simulink model "heatdrive_ecc_coupled_se21"  (R2025b)
settings: Solver=ode23t  StartTime=0.0  StopTime=10  FixedStep=0.1  MaxStep=0.4  RelTol=1e-2  AbsTol=1e-3
values from neighbouring files (symbols this model uses):
  cold_load_heat_W = 0.0    (= 0)    [Build_Simulink_Exchange_Params.m]
  cold_load_T_init = get_stage_field(stage_config, 'cold_load_T_in', get_stage_field(stage_config,          'chip_T_in', get_option_field(exchange_options, 'cold_load_T_init', get_option_field(exchange_options, 'chip_T_init', 293.0))))    [Build_Simulink_Exchange_Params.m]    (also in Create_Simulink_Exchange_Runtime.m = get_option_field(options, 'cold_load_T_init',          get_o)
  cold_sink_T_init = get_stage_field(stage_config, 'cold_sink_T_in', get_option_field(exchange_options, 'cold_sink_T_init', 293.0))    [Build_Simulink_Exchange_Params.m]    (also in Create_Simulink_Exchange_Runtime.m = get_option_field(options, 'cold_sink_T_init', ambient_T_init)
  hot_sink_T_init = get_stage_field(stage_config, 'hot_sink_T_in', get_option_field(exchange_options, 'hot_sink_T_init', 293.0))    [Build_Simulink_Exchange_Params.m]    (also in Create_Simulink_Exchange_Runtime.m = get_option_field(options, 'hot_sink_T_init', ambient_T_init))
  mdot_cooldown_source_kgps = mdot_target_kgps    [Build_Simulink_Exchange_Params.m]
  mdot_hold_source_kgps = mdot_target_kgps    [Build_Simulink_Exchange_Params.m]
  pressure_pi_bias_MPa = pressure_pi_dp_guess_MPa    [Build_Simulink_Exchange_Params.m]
  pressure_pi_error_filter_tau_s = max(get_option_field(exchange_options, 'pressure_pi_error_filter_tau_s', 0.002), 1.0e-5)    [Build_Simulink_Exchange_Params.m]
  pressure_pi_error_normalization_gain_kgps_inv = 1.0    (= 1)    [Build_Simulink_Exchange_Params.m]
  pressure_pi_max_MPa = pressure_pi_dp_guess_MPa + pressure_pi_margin_MPa    [Build_Simulink_Exchange_Params.m]
  shex_sink_T_init = get_option_field(exchange_options, 'shex_sink_T_init', hot_sink_T_init)    [Build_Simulink_Exchange_Params.m]
undefined symbols (not defined in the file or in its folder): constitutive_sample_time_s, constitutive_state21_initial, se_constitutive_T21_initial, se_pressure_integrator_max_MPa, se_pressure_pi_ki_MPa_per_kgps_s, se_pressure_pi_kp_MPa_per_kgps, se_pressure_pi_min_MPa, se_solver_T_init_21_internal, se_stage2_pressure_integrator_min_MPa, se_stage4_pressure_integrator_min_MPa, sma_constitutive_T21_initial, sma_mdot_stage1_source_kgps, sma_mdot_stage3_source_kgps, sma_pressure_integrator_max_MPa, sma_pressure_integrator_min_MPa, sma_pressure_pi_ki_MPa_per_kgps_s, sma_pressure_pi_kp_MPa_per_kgps, sma_pressure_pi_min_MPa, sma_solver_T_init_21_internal
libraries: fl_lib x484, nesl_utility x232, SimscapeFluids_lib x20
(part 5 of 8)

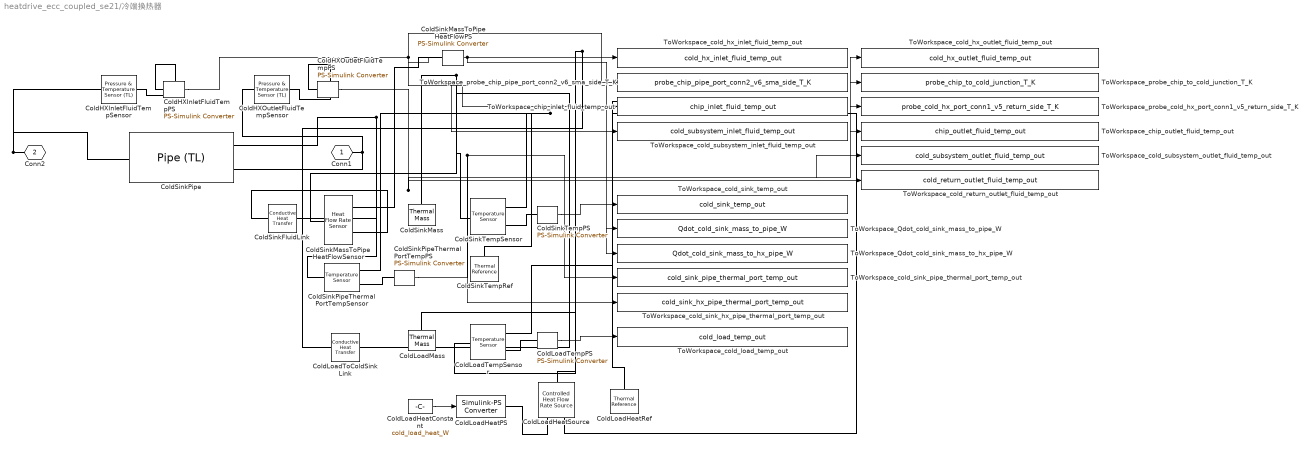
== system heatdrive_ecc_coupled_se21/冷端换热器 ==
  ColdHXInletFluidTempPS : nesl_utility/PS-Simulink Converter  PhysicalDomain=network_engine_domain  SubClassName=ps_output  LeftPortType=input  RightPortType=output  PseudoPeriodic=off  Frequencies=[]  VectorFormat=1-D array  Unit=K  AffineConversion=off
  ColdHXInletFluidTempSensor : fl_lib/Thermal Liquid/Sensors/Pressure & Temperature Sensor (TL)  reference=foundation.enum.MeasurementReference.absolute  pressure=false  pressure_spec=foundation.enum.PressureMeasementSpec.Absolute  temperature=true
      settings: InternalSimscapePortConfiguration="{\"Bottom\":[{\"id\":\"T\",\"label\":\"T\",\"type\":\"output\"}],\"Left\":[{\"id\":\"A\",\"label\":\"A\",\"type\":\"foundation.thermal_liquid.thermal_liquid\"}],\"Right\":[],\"Top\":[]}"
  ColdHXOutletFluidTempPS : nesl_utility/PS-Simulink Converter  PhysicalDomain=network_engine_domain  SubClassName=ps_output  LeftPortType=input  RightPortType=output  PseudoPeriodic=off  Frequencies=[]  VectorFormat=1-D array  Unit=K  AffineConversion=off
  ColdHXOutletFluidTempSensor : fl_lib/Thermal Liquid/Sensors/Pressure & Temperature Sensor (TL)  reference=foundation.enum.MeasurementReference.absolute  pressure=false  pressure_spec=foundation.enum.PressureMeasementSpec.Absolute  temperature=true
      settings: InternalSimscapePortConfiguration="{\"Bottom\":[{\"id\":\"T\",\"label\":\"T\",\"type\":\"output\"}],\"Left\":[{\"id\":\"A\",\"label\":\"A\",\"type\":\"foundation.thermal_liquid.thermal_liquid\"}],\"Right\":[],\"Top\":[]}"
  ColdLoadHeatConstant : Constant  Value=cold_load_heat_W
  ColdLoadHeatPS : nesl_utility/Simulink-PS Converter  PhysicalDomain=network_engine_domain  SubClassName=ps_input  LeftPortType=input  RightPortType=output  PseudoPeriodic=off  Frequencies=[]  NoiseDistribution=none  NoiseParameters=[]  Unit=W  AffineConversion=off  FilteringAndDerivatives=provide  SimscapeFilterOrder=1  InputFilterTimeConstant=0.001  UdotUserProvided=0
  ColdLoadHeatRef : fl_lib/Thermal/Thermal Elements/Thermal Reference
  ColdLoadHeatSource : fl_lib/Thermal/Thermal Sources/Controlled Heat Flow Rate Source
  ColdLoadMass : fl_lib/Thermal/Thermal Elements/Thermal Mass  mass_type=foundation.enum.constant_variable.constant  mass=cold_load_mass_kg kg  sp_heat=thermal_mass_cp_ref J/(K*kg)  mass_min=1e-6 kg  num_ports=foundation.enum.numPorts2.one  m_specify=off  m_priority=High  m=1 kg  m_nominal_specify=off  m_nominal_value=1  m_nominal_unit=kg  T_specify=on  T_priority=High  T=cold_load_T_init K  T_nominal_specify=off  T_nominal_value=1  T_nominal_unit=K  Q_specify=off  Q_priority=None  Q=0 W  Q_nominal_specify=off  Q_nominal_value=1  Q_nominal_unit=W
  ColdLoadTempPS : nesl_utility/PS-Simulink Converter  PhysicalDomain=network_engine_domain  SubClassName=ps_output  LeftPortType=input  RightPortType=output  PseudoPeriodic=off  Frequencies=[]  VectorFormat=1-D array  Unit=K  AffineConversion=off
  ColdLoadTempSensor : fl_lib/Thermal/Thermal Sensors/Temperature Sensor  temperature_measure=foundation.enum.MeasurementReference.difference
  ColdLoadToColdSinkLink : fl_lib/Thermal/Thermal Elements/Conductive Heat Transfer  thermal_type=foundation.enum.ConstantVariableTabulated.Constant  wall_geometry=foundation.enum.ConductionWallGeometry.Planar  area=1 m^2  thickness=1 m  d_in=0.05 m  d_out=0.1 m  L=1 m  th_cond_min=10 W/(K*m)  th_cond=cold_load_to_cold_sink_G_W_per_K W/(K*m)  th_cond_TLU=[413, 401, 392, 383, 371, 357, 342] W/(K*m)  temp_TLU=[200, 273, 400, 600, 800, 1000, 1200] K  T_specify=off  T_priority=None  T=0 K  T_nominal_specify=off  T_nominal_value=1  T_nominal_unit=K  Q_specify=off  Q_priority=None  Q=0 W  Q_nominal_specify=off  Q_nominal_value=1  Q_nominal_unit=W
  ColdSinkFluidLink : fl_lib/Thermal/Thermal Elements/Conductive Heat Transfer  thermal_type=foundation.enum.ConstantVariableTabulated.Constant  wall_geometry=foundation.enum.ConductionWallGeometry.Planar  area=1 m^2  thickness=1 m  d_in=0.05 m  d_out=0.1 m  L=1 m  th_cond_min=10 W/(K*m)  th_cond=cold_sink_fluid_G_W_per_K W/(K*m)  th_cond_TLU=[413, 401, 392, 383, 371, 357, 342] W/(K*m)  temp_TLU=[200, 273, 400, 600, 800, 1000, 1200] K  T_specify=off  T_priority=None  T=0 K  T_nominal_specify=off  T_nominal_value=1  T_nominal_unit=K  Q_specify=off  Q_priority=None  Q=0 W  Q_nominal_specify=off  Q_nominal_value=1  Q_nominal_unit=W
  ColdSinkMass : fl_lib/Thermal/Thermal Elements/Thermal Mass  mass_type=foundation.enum.constant_variable.constant  mass=cold_sink_mass_kg kg  sp_heat=thermal_mass_cp_ref J/(K*kg)  mass_min=1e-6 kg  num_ports=foundation.enum.numPorts2.one  m_specify=off  m_priority=High  m=1 kg  m_nominal_specify=off  m_nominal_value=1  m_nominal_unit=kg  T_specify=on  T_priority=High  T=cold_sink_T_init K  T_nominal_specify=off  T_nominal_value=1  T_nominal_unit=K  Q_specify=off  Q_priority=None  Q=0 W  Q_nominal_specify=off  Q_nominal_value=1  Q_nominal_unit=W
  ColdSinkMassToPipeHeatFlowPS : nesl_utility/PS-Simulink Converter  PhysicalDomain=network_engine_domain  SubClassName=ps_output  LeftPortType=input  RightPortType=output  PseudoPeriodic=off  Frequencies=[]  VectorFormat=1-D array  Unit=W  AffineConversion=off
  ColdSinkMassToPipeHeatFlowSensor : fl_lib/Thermal/Thermal Sensors/Heat Flow Rate Sensor
  ColdSinkPipe : fl_lib/Thermal Liquid/Elements/Pipe (TL)  length=cold_pipe_or_CHEX_length_m m  area=pipe_fa m^2  Dh=D_e m  length_add=0 m  roughness=15e-6 m  Re_lam=2000  Re_tur=4000  shape_factor=64  Nu_lam=nuh  dynamic_compressibility=false  inertia=false  p0=1 MPa  T0=cold_side_fluid_T_init K  mdot0=0 kg/s  p_nominal=1 MPa  T_nominal=293.15 K
  ColdSinkPipeThermalPortTempPS : nesl_utility/PS-Simulink Converter  PhysicalDomain=network_engine_domain  SubClassName=ps_output  LeftPortType=input  RightPortType=output  PseudoPeriodic=off  Frequencies=[]  VectorFormat=1-D array  Unit=K  AffineConversion=off
  ColdSinkPipeThermalPortTempSensor : fl_lib/Thermal/Thermal Sensors/Temperature Sensor  temperature_measure=foundation.enum.MeasurementReference.difference
  ColdSinkTempPS : nesl_utility/PS-Simulink Converter  PhysicalDomain=network_engine_domain  SubClassName=ps_output  LeftPortType=input  RightPortType=output  PseudoPeriodic=off  Frequencies=[]  VectorFormat=1-D array  Unit=K  AffineConversion=off
  ColdSinkTempRef : fl_lib/Thermal/Thermal Elements/Thermal Reference
  ColdSinkTempSensor : fl_lib/Thermal/Thermal Sensors/Temperature Sensor  temperature_measure=foundation.enum.MeasurementReference.difference
  ToWorkspace_Qdot_cold_sink_mass_to_hx_pipe_W : ToWorkspace  VariableName=Qdot_cold_sink_mass_to_hx_pipe_W  SaveFormat=Structure With Time  SampleTime=-1
  ToWorkspace_Qdot_cold_sink_mass_to_pipe_W : ToWorkspace  VariableName=Qdot_cold_sink_mass_to_pipe_W  SaveFormat=Structure With Time  SampleTime=-1
  ToWorkspace_chip_inlet_fluid_temp_out : ToWorkspace  VariableName=chip_inlet_fluid_temp_out  SaveFormat=Structure With Time  SampleTime=-1
  ToWorkspace_chip_outlet_fluid_temp_out : ToWorkspace  VariableName=chip_outlet_fluid_temp_out  SaveFormat=Structure With Time  SampleTime=-1
  ToWorkspace_cold_hx_inlet_fluid_temp_out : ToWorkspace  VariableName=cold_hx_inlet_fluid_temp_out  SaveFormat=Structure With Time  SampleTime=-1
  ToWorkspace_cold_hx_outlet_fluid_temp_out : ToWorkspace  VariableName=cold_hx_outlet_fluid_temp_out  SaveFormat=Structure With Time  SampleTime=-1
  ToWorkspace_cold_load_temp_out : ToWorkspace  VariableName=cold_load_temp_out  SaveFormat=Structure With Time  SampleTime=-1
  ToWorkspace_cold_return_outlet_fluid_temp_out : ToWorkspace  VariableName=cold_return_outlet_fluid_temp_out  SaveFormat=Structure With Time  SampleTime=-1
  ToWorkspace_cold_sink_hx_pipe_thermal_port_temp_out : ToWorkspace  VariableName=cold_sink_hx_pipe_thermal_port_temp_out  SaveFormat=Structure With Time  SampleTime=-1
  ToWorkspace_cold_sink_pipe_thermal_port_temp_out : ToWorkspace  VariableName=cold_sink_pipe_thermal_port_temp_out  SaveFormat=Structure With Time  SampleTime=-1
  ToWorkspace_cold_sink_temp_out : ToWorkspace  VariableName=cold_sink_temp_out  SaveFormat=Structure With Time  SampleTime=-1
  ToWorkspace_cold_subsystem_inlet_fluid_temp_out : ToWorkspace  VariableName=cold_subsystem_inlet_fluid_temp_out  SaveFormat=Structure With Time  SampleTime=-1
  ToWorkspace_cold_subsystem_outlet_fluid_temp_out : ToWorkspace  VariableName=cold_subsystem_outlet_fluid_temp_out  SaveFormat=Structure With Time  SampleTime=-1
  ToWorkspace_probe_chip_pipe_port_conn2_v6_sma_side_T_K : ToWorkspace  VariableName=probe_chip_pipe_port_conn2_v6_sma_side_T_K  SaveFormat=Structure With Time  SampleTime=-1
  ToWorkspace_probe_chip_to_cold_junction_T_K : ToWorkspace  VariableName=probe_chip_to_cold_junction_T_K  SaveFormat=Structure With Time  SampleTime=-1
  ToWorkspace_probe_cold_hx_port_conn1_v5_return_side_T_K : ToWorkspace  VariableName=probe_cold_hx_port_conn1_v5_return_side_T_K  SaveFormat=Structure With Time  SampleTime=-1
  Conn1 : PMIOPort  Side=Right
  Conn2 : PMIOPort  Port=2  Side=Left
  wires:
  ColdSinkMassToPipeHeatFlowPS/1 -> ToWorkspace_Qdot_cold_sink_mass_to_hx_pipe_W/1, ToWorkspace_Qdot_cold_sink_mass_to_pipe_W/1
  ColdSinkPipeThermalPortTempPS/1 -> ToWorkspace_cold_sink_hx_pipe_thermal_port_temp_out/1, ToWorkspace_cold_sink_pipe_thermal_port_temp_out/1
  ColdLoadTempPS/1 -> ToWorkspace_cold_load_temp_out/1
  ColdLoadHeatConstant/1 -> ColdLoadHeatPS/1
  ColdSinkTempPS/1 -> ToWorkspace_cold_sink_temp_out/1
  ColdHXInletFluidTempPS/1 -> ToWorkspace_cold_hx_inlet_fluid_temp_out/1, ToWorkspace_probe_chip_pipe_port_conn2_v6_sma_side_T_K/1, ToWorkspace_chip_inlet_fluid_temp_out/1, ToWorkspace_cold_subsystem_inlet_fluid_temp_out/1
  ColdHXOutletFluidTempPS/1 -> ToWorkspace_cold_hx_outlet_fluid_temp_out/1, ToWorkspace_probe_chip_to_cold_junction_T_K/1, ToWorkspace_probe_cold_hx_port_conn1_v5_return_side_T_K/1, ToWorkspace_chip_outlet_fluid_temp_out/1, ToWorkspace_cold_subsystem_outlet_fluid_temp_out/1, ToWorkspace_cold_return_outlet_fluid_temp_out/1
  connections:
  Conn2/RConn1 -- ColdSinkPipe/RConn1 -- ColdHXInletFluidTempSensor/LConn1
  Conn1/RConn1 -- ColdSinkPipe/LConn1 -- ColdHXOutletFluidTempSensor/LConn1
  ColdLoadToColdSinkLink/LConn1 -- ColdLoadMass/LConn1 -- ColdLoadTempSensor/LConn1 -- ColdLoadHeatSource/LConn1
  ColdLoadToColdSinkLink/RConn1 -- ColdSinkMassToPipeHeatFlowSensor/LConn1 -- ColdSinkMass/LConn1 -- ColdSinkTempSensor/LConn1
  ColdLoadHeatRef/LConn1 -- ColdLoadTempSensor/RConn1 -- ColdLoadHeatSource/RConn2
  ColdLoadTempSensor/RConn2 -- ColdLoadTempPS/LConn1
  ColdLoadHeatPS/RConn1 -- ColdLoadHeatSource/RConn1
  ColdSinkMassToPipeHeatFlowSensor/RConn2 -- ColdSinkFluidLink/LConn1
  ColdSinkMassToPipeHeatFlowSensor/RConn1 -- ColdSinkMassToPipeHeatFlowPS/LConn1
  ColdSinkPipe/LConn2 -- ColdSinkFluidLink/RConn1 -- ColdSinkPipeThermalPortTempSensor/LConn1
  ColdSinkTempRef/LConn1 -- ColdSinkPipeThermalPortTempSensor/RConn1 -- ColdSinkTempSensor/RConn1
  ColdSinkPipeThermalPortTempSensor/RConn2 -- ColdSinkPipeThermalPortTempPS/LConn1
  ColdSinkTempSensor/RConn2 -- ColdSinkTempPS/LConn1
  ColdHXInletFluidTempSensor/RConn1 -- ColdHXInletFluidTempPS/LConn1
  ColdHXOutletFluidTempSensor/RConn1 -- ColdHXOutletFluidTempPS/LConn1

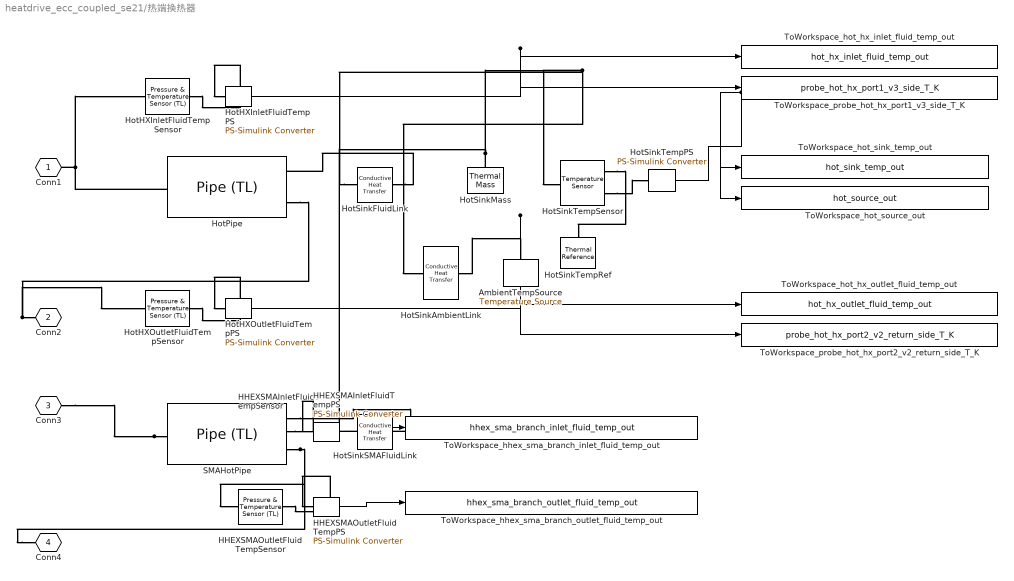
== system heatdrive_ecc_coupled_se21/热端换热器 ==
  AmbientTempSource : fl_lib/Thermal/Thermal Sources/Temperature Source  temperature=ambient_T_init K
  HHEXSMAInletFluidTempPS : nesl_utility/PS-Simulink Converter  PhysicalDomain=network_engine_domain  SubClassName=ps_output  LeftPortType=input  RightPortType=output  PseudoPeriodic=off  Frequencies=[]  VectorFormat=1-D array  Unit=K  AffineConversion=off
  HHEXSMAInletFluidTempSensor : fl_lib/Thermal Liquid/Sensors/Pressure & Temperature Sensor (TL)  reference=foundation.enum.MeasurementReference.absolute  pressure=false  pressure_spec=foundation.enum.PressureMeasementSpec.Absolute  temperature=true
      settings: InternalSimscapePortConfiguration="{\"Bottom\":[{\"id\":\"T\",\"label\":\"T\",\"type\":\"output\"}],\"Left\":[{\"id\":\"A\",\"label\":\"A\",\"type\":\"foundation.thermal_liquid.thermal_liquid\"}],\"Right\":[],\"Top\":[]}"
  HHEXSMAOutletFluidTempPS : nesl_utility/PS-Simulink Converter  PhysicalDomain=network_engine_domain  SubClassName=ps_output  LeftPortType=input  RightPortType=output  PseudoPeriodic=off  Frequencies=[]  VectorFormat=1-D array  Unit=K  AffineConversion=off
  HHEXSMAOutletFluidTempSensor : fl_lib/Thermal Liquid/Sensors/Pressure & Temperature Sensor (TL)  reference=foundation.enum.MeasurementReference.absolute  pressure=false  pressure_spec=foundation.enum.PressureMeasementSpec.Absolute  temperature=true
      settings: InternalSimscapePortConfiguration="{\"Bottom\":[{\"id\":\"T\",\"label\":\"T\",\"type\":\"output\"}],\"Left\":[{\"id\":\"A\",\"label\":\"A\",\"type\":\"foundation.thermal_liquid.thermal_liquid\"}],\"Right\":[],\"Top\":[]}"
  HotHXInletFluidTempPS : nesl_utility/PS-Simulink Converter  PhysicalDomain=network_engine_domain  SubClassName=ps_output  LeftPortType=input  RightPortType=output  PseudoPeriodic=off  Frequencies=[]  VectorFormat=1-D array  Unit=K  AffineConversion=off
  HotHXInletFluidTempSensor : fl_lib/Thermal Liquid/Sensors/Pressure & Temperature Sensor (TL)  reference=foundation.enum.MeasurementReference.absolute  pressure=false  pressure_spec=foundation.enum.PressureMeasementSpec.Absolute  temperature=true
      settings: InternalSimscapePortConfiguration="{\"Bottom\":[{\"id\":\"T\",\"label\":\"T\",\"type\":\"output\"}],\"Left\":[{\"id\":\"A\",\"label\":\"A\",\"type\":\"foundation.thermal_liquid.thermal_liquid\"}],\"Right\":[],\"Top\":[]}"
  HotHXOutletFluidTempPS : nesl_utility/PS-Simulink Converter  PhysicalDomain=network_engine_domain  SubClassName=ps_output  LeftPortType=input  RightPortType=output  PseudoPeriodic=off  Frequencies=[]  VectorFormat=1-D array  Unit=K  AffineConversion=off
  HotHXOutletFluidTempSensor : fl_lib/Thermal Liquid/Sensors/Pressure & Temperature Sensor (TL)  reference=foundation.enum.MeasurementReference.absolute  pressure=false  pressure_spec=foundation.enum.PressureMeasementSpec.Absolute  temperature=true
      settings: InternalSimscapePortConfiguration="{\"Bottom\":[{\"id\":\"T\",\"label\":\"T\",\"type\":\"output\"}],\"Left\":[{\"id\":\"A\",\"label\":\"A\",\"type\":\"foundation.thermal_liquid.thermal_liquid\"}],\"Right\":[],\"Top\":[]}"
  HotPipe : fl_lib/Thermal Liquid/Elements/Pipe (TL)  length=tube_l m  area=pipe_fa m^2  Dh=D_e m  length_add=0 m  roughness=15e-6 m  Re_lam=2000  Re_tur=4000  shape_factor=64  Nu_lam=nuh  dynamic_compressibility=false  inertia=false  p0=1 MPa  T0=hot_side_fluid_T_init K  mdot0=0 kg/s  p_nominal=1 MPa  T_nominal=293.15 K
  HotSinkAmbientLink : fl_lib/Thermal/Thermal Elements/Conductive Heat Transfer  thermal_type=foundation.enum.ConstantVariableTabulated.Constant  wall_geometry=foundation.enum.ConductionWallGeometry.Planar  area=1 m^2  thickness=1 m  d_in=0.05 m  d_out=0.1 m  L=1 m  th_cond_min=10 W/(K*m)  th_cond=hot_sink_ambient_G_W_per_K W/(K*m)  th_cond_TLU=[413, 401, 392, 383, 371, 357, 342] W/(K*m)  temp_TLU=[200, 273, 400, 600, 800, 1000, 1200] K  T_specify=off  T_priority=None  T=0 K  T_nominal_specify=off  T_nominal_value=1  T_nominal_unit=K  Q_specify=off  Q_priority=None  Q=0 W  Q_nominal_specify=off  Q_nominal_value=1  Q_nominal_unit=W
  HotSinkFluidLink : fl_lib/Thermal/Thermal Elements/Conductive Heat Transfer  thermal_type=foundation.enum.ConstantVariableTabulated.Constant  wall_geometry=foundation.enum.ConductionWallGeometry.Planar  area=1 m^2  thickness=1 m  d_in=0.05 m  d_out=0.1 m  L=1 m  th_cond_min=10 W/(K*m)  th_cond=hot_sink_fluid_G_W_per_K W/(K*m)  th_cond_TLU=[413, 401, 392, 383, 371, 357, 342] W/(K*m)  temp_TLU=[200, 273, 400, 600, 800, 1000, 1200] K  T_specify=off  T_priority=None  T=0 K  T_nominal_specify=off  T_nominal_value=1  T_nominal_unit=K  Q_specify=off  Q_priority=None  Q=0 W  Q_nominal_specify=off  Q_nominal_value=1  Q_nominal_unit=W
  HotSinkMass : fl_lib/Thermal/Thermal Elements/Thermal Mass  mass_type=foundation.enum.constant_variable.constant  mass=hot_sink_mass_kg kg  sp_heat=thermal_mass_cp_ref J/(K*kg)  mass_min=1e-6 kg  num_ports=foundation.enum.numPorts2.one  m_specify=off  m_priority=High  m=1 kg  m_nominal_specify=off  m_nominal_value=1  m_nominal_unit=kg  T_specify=on  T_priority=High  T=hot_sink_T_init K  T_nominal_specify=off  T_nominal_value=1  T_nominal_unit=K  Q_specify=off  Q_priority=None  Q=0 W  Q_nominal_specify=off  Q_nominal_value=1  Q_nominal_unit=W
  HotSinkSMAFluidLink : fl_lib/Thermal/Thermal Elements/Conductive Heat Transfer  thermal_type=foundation.enum.ConstantVariableTabulated.Constant  wall_geometry=foundation.enum.ConductionWallGeometry.Planar  area=1 m^2  thickness=1 m  d_in=0.05 m  d_out=0.1 m  L=1 m  th_cond_min=10 W/(K*m)  th_cond=hot_sink_sma_fluid_G_W_per_K W/(K*m)  th_cond_TLU=[413, 401, 392, 383, 371, 357, 342] W/(K*m)  temp_TLU=[200, 273, 400, 600, 800, 1000, 1200] K  T_specify=off  T_priority=None  T=0 K  T_nominal_specify=off  T_nominal_value=1  T_nominal_unit=K  Q_specify=off  Q_priority=None  Q=0 W  Q_nominal_specify=off  Q_nominal_value=1  Q_nominal_unit=W
  HotSinkTempPS : nesl_utility/PS-Simulink Converter  PhysicalDomain=network_engine_domain  SubClassName=ps_output  LeftPortType=input  RightPortType=output  PseudoPeriodic=off  Frequencies=[]  VectorFormat=1-D array  Unit=K  AffineConversion=off
  HotSinkTempRef : fl_lib/Thermal/Thermal Elements/Thermal Reference
  HotSinkTempSensor : fl_lib/Thermal/Thermal Sensors/Temperature Sensor  temperature_measure=foundation.enum.MeasurementReference.difference
  SMAHotPipe : fl_lib/Thermal Liquid/Elements/Pipe (TL)  length=tube_l m  area=sma_pipe_fa m^2  Dh=D_e m  length_add=0 m  roughness=15e-6 m  Re_lam=2000  Re_tur=4000  shape_factor=64  Nu_lam=nuh  dynamic_compressibility=false  inertia=false  p0=1 MPa  T0=hot_side_fluid_T_init K  mdot0=0 kg/s  p_nominal=1 MPa  T_nominal=293.15 K
  ToWorkspace_hhex_sma_branch_inlet_fluid_temp_out : ToWorkspace  VariableName=hhex_sma_branch_inlet_fluid_temp_out  SaveFormat=Structure With Time  SampleTime=-1
  ToWorkspace_hhex_sma_branch_outlet_fluid_temp_out : ToWorkspace  VariableName=hhex_sma_branch_outlet_fluid_temp_out  SaveFormat=Structure With Time  SampleTime=-1
  ToWorkspace_hot_hx_inlet_fluid_temp_out : ToWorkspace  VariableName=hot_hx_inlet_fluid_temp_out  SaveFormat=Structure With Time  SampleTime=-1
  ToWorkspace_hot_hx_outlet_fluid_temp_out : ToWorkspace  VariableName=hot_hx_outlet_fluid_temp_out  SaveFormat=Structure With Time  SampleTime=-1
  ToWorkspace_hot_sink_temp_out : ToWorkspace  VariableName=hot_sink_temp_out  SaveFormat=Structure With Time  SampleTime=-1
  ToWorkspace_hot_source_out : ToWorkspace  VariableName=hot_source_out  SaveFormat=Structure With Time  SampleTime=-1
  ToWorkspace_probe_hot_hx_port1_v3_side_T_K : ToWorkspace  VariableName=probe_hot_hx_port1_v3_side_T_K  SaveFormat=Structure With Time  SampleTime=-1
  ToWorkspace_probe_hot_hx_port2_v2_return_side_T_K : ToWorkspace  VariableName=probe_hot_hx_port2_v2_return_side_T_K  SaveFormat=Structure With Time  SampleTime=-1
  Conn1 : PMIOPort  Side=Right
  Conn2 : PMIOPort  Port=2  Side=Left
  Conn3 : PMIOPort  Port=3  Side=Right
  Conn4 : PMIOPort  Port=4  Side=Left
  wires:
  HotSinkTempPS/1 -> ToWorkspace_hot_sink_temp_out/1, ToWorkspace_hot_source_out/1
  HotHXInletFluidTempPS/1 -> ToWorkspace_hot_hx_inlet_fluid_temp_out/1, ToWorkspace_probe_hot_hx_port1_v3_side_T_K/1
  HotHXOutletFluidTempPS/1 -> ToWorkspace_hot_hx_outlet_fluid_temp_out/1, ToWorkspace_probe_hot_hx_port2_v2_return_side_T_K/1
  HHEXSMAInletFluidTempPS/1 -> ToWorkspace_hhex_sma_branch_inlet_fluid_temp_out/1
  HHEXSMAOutletFluidTempPS/1 -> ToWorkspace_hhex_sma_branch_outlet_fluid_temp_out/1
  connections:
  Conn1/RConn1 -- HotPipe/RConn1 -- HotHXInletFluidTempSensor/LConn1
  Conn2/RConn1 -- HotPipe/LConn1 -- HotHXOutletFluidTempSensor/LConn1
  HotSinkFluidLink/LConn1 -- HotSinkMass/LConn1 -- HotSinkSMAFluidLink/LConn1 -- HotSinkTempSensor/LConn1 -- HotSinkAmbientLink/LConn1
  HotSinkFluidLink/RConn1 -- HotPipe/LConn2
  HotSinkTempSensor/RConn1 -- HotSinkTempRef/LConn1
  HotSinkTempSensor/RConn2 -- HotSinkTempPS/LConn1
  HotSinkAmbientLink/RConn1 -- AmbientTempSource/LConn1
  HotHXInletFluidTempSensor/RConn1 -- HotHXInletFluidTempPS/LConn1
  HotHXOutletFluidTempSensor/RConn1 -- HotHXOutletFluidTempPS/LConn1
  SMAHotPipe/LConn2 -- HotSinkSMAFluidLink/RConn1
  SMAHotPipe/RConn1 -- Conn3/RConn1 -- HHEXSMAInletFluidTempSensor/LConn1
  HHEXSMAInletFluidTempSensor/RConn1 -- HHEXSMAInletFluidTempPS/LConn1
  Conn4/RConn1 -- SMAHotPipe/LConn1 -- HHEXSMAOutletFluidTempSensor/LConn1
  HHEXSMAOutletFluidTempSensor/RConn1 -- HHEXSMAOutletFluidTempPS/LConn1
